simulink model "Shaddad_Perception"  (R2026b)
undefined symbols (not defined in the file): P, sens_per_prior_map, sens_per_prm, Ts
libraries: simulink x7, ros2lib x3, dspstat3 x1
settings Model: Creator=aomar  LastModifiedBy=aomar

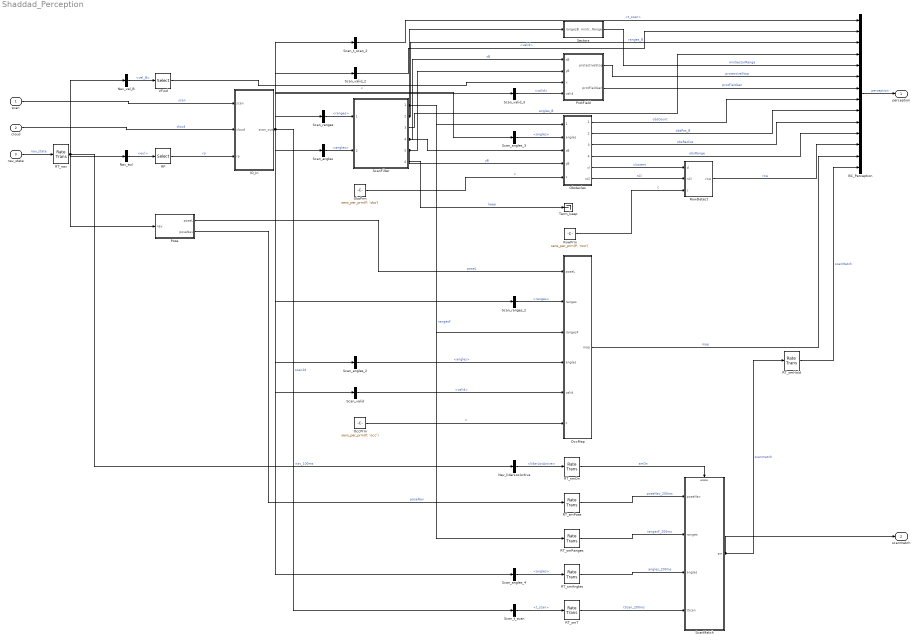
== system Shaddad_Perception ==
  scan : Inport  OutDataTypeStr=Bus: Bus_LidarScanRaw  SampleTime=Ts.lidar  BusOutputAsStruct=on
  cloud : Inport  Port=2  OutDataTypeStr=Bus: Bus_LidarCloudRaw  SampleTime=Ts.lidar  BusOutputAsStruct=on
  nav_state : Inport  Port=3  OutDataTypeStr=Bus: Bus_NavState  SampleTime=Ts.nav  BusOutputAsStruct=on
  BC_Perception : BusCreator  Inputs=14  OutDataTypeStr=Bus: Bus_Perception  NonVirtualBus=on
      settings: InheritFromInputs=off
  IO_In : Subsystem  Variant=on
  Nav_eul : BusSelector  OutputSignals=eul
  Nav_lidarLocActive : BusSelector  OutputSignals=lidarLocActive
  Nav_vel_B : BusSelector  OutputSignals=vel_B
  ObsPrm : Constant  Value=sens_per_prm(P, 'obs')
  Obstacles : MATLAB Function  TreatAsAtomicUnit=on
  OccMap : MATLAB Function  TreatAsAtomicUnit=on
  OccPrm : Constant  Value=sens_per_prm(P, 'occ')
  Pose : Subsystem  Description=poseL = [x + rLx cos psi - rLy sin psi, y + rLx sin psi + rLy cos psi, psi + psiL]; poseNav = [x y psi].
  ProtField : Subsystem  Description=Protective field (sensors spec 3.7): length protL0 + protKv |v|, width protW; the front field ahead of x = protXF (front of the body or of the fitted implement) when v > -protVBoth, the rear field behind x = protXR (rear of the body or implement) when v < protVBoth (both at standstill); a field stops when any kept point lies inside. Scan lost or stale (critfix R-02): on an invalid scan the last valid field result is held for up to protNStale scans, then protectiveStop is true until a valid scan arrives; true from the start until the first valid scan.
  RP : Selector  InputPortWidth=3  IndexOptions=Index vector (dialog)  Indices=[3 2]  OutputSizes=1
  RT_nav : RateTransition  OutPortSampleTime=Ts.perception
  RT_smAngles : RateTransition  OutPortSampleTime=Ts.scanmatch
  RT_smHold : RateTransition  InitialCondition=P.ic.Bus_ScanMatchMeas  OutPortSampleTime=Ts.perception
  RT_smOn : RateTransition  OutPortSampleTime=Ts.scanmatch
  RT_smPose : RateTransition  OutPortSampleTime=Ts.scanmatch
  RT_smRanges : RateTransition  OutPortSampleTime=Ts.scanmatch
  RT_smT : RateTransition  OutPortSampleTime=Ts.scanmatch
  RowDetect : MATLAB Function  TreatAsAtomicUnit=on
  RowPrm : Constant  Value=sens_per_prm(P, 'row')
  ScanFilter : Subsystem  ReferencedSubsystem=sens_scan_filter
  ScanMatch : Subsystem  Description=Enabled at 0.2 s while nav_state.lidarLocActive (D55); output reset to P.ic.Bus_ScanMatchMeas (valid false) while disabled.  TreatAsAtomicUnit=on
  Scan_angles : BusSelector  OutputSignals=angles
  Scan_angles_2 : BusSelector  OutputSignals=angles
  Scan_angles_3 : BusSelector  OutputSignals=angles
  Scan_angles_4 : BusSelector  OutputSignals=angles
  Scan_ranges : BusSelector  OutputSignals=ranges
  Scan_ranges_2 : BusSelector  OutputSignals=ranges
  Scan_t_scan : BusSelector  OutputSignals=t_scan
  Scan_t_scan_2 : BusSelector  OutputSignals=t_scan
  Scan_valid : BusSelector  OutputSignals=valid
  Scan_valid_2 : BusSelector  OutputSignals=valid
  Scan_valid_3 : BusSelector  OutputSignals=valid
  Sectors : Subsystem  Description=8 x 45 deg sector minima of ranges_B (sector j covers sensor beams -22 + 45 (j-1) ... +22 + 45 (j-1) deg, CCW): NaN -> Inf, Selector P.sensors.per.secIdx, Reshape [45 8], dspstat3/Minimum per column, empty sector -> NaN.
  Term_keep : Terminator
  VFwd : Selector  InputPortWidth=3  IndexOptions=Index vector (dialog)  Indices=1  OutputSizes=1
  perception : Outport  OutDataTypeStr=Bus: Bus_Perception  SampleTime=Ts.perception  BusOutputAsStruct=on
  scanmatch : Outport  Port=2  OutDataTypeStr=Bus: Bus_ScanMatchMeas  SampleTime=Ts.scanmatch  BusOutputAsStruct=on
  wires:
  scan/1 -> IO_In/1(scan)  "scan"
  cloud/1 -> IO_In/2(cloud)  "cloud"
  nav_state/1 -> RT_nav/1  "nav_state"
  RT_nav/1 -> Nav_lidarLocActive/1, Nav_vel_B/1, Pose/1(nav), Nav_eul/1  "nav_100ms"
  Nav_vel_B/1 -> VFwd/1  "<vel_B>"
  Nav_eul/1 -> RP/1  "<eul>"
  VFwd/1 -> ProtField/3(v)  "v"
  RP/1 -> IO_In/3(rp)  "rp"
  Pose/1(poseL) -> OccMap/1(poseL)  "poseL"
  Pose/2(poseNav) -> RT_smPose/1  "poseNav"
  IO_In/1(scan_out) -> Scan_t_scan/1, Scan_angles_4/1, Scan_valid/1, Scan_angles_2/1, Scan_ranges_2/1, Scan_t_scan_2/1, Scan_valid_2/1, Scan_valid_3/1, Scan_angles/1, Scan_ranges/1, Scan_angles_3/1  "scan2d"
  Scan_ranges/1 -> ScanFilter/1  "<ranges>"
  Scan_angles/1 -> ScanFilter/2  "<angles>"
  Scan_t_scan_2/1 -> BC_Perception/1  "<t_scan>"
  Scan_valid_2/1 -> BC_Perception/2  "<valid>"
  Scan_angles_2/1 -> OccMap/4(angles)  "<angles>"
  Scan_valid/1 -> OccMap/5(valid)  "<valid>"
  ObsPrm/1 -> Obstacles/5(c)  "c"
  OccPrm/1 -> OccMap/6(c)  "c"
  ScanFilter/3 -> BC_Perception/4  "angles_B"
  ScanFilter/6 -> Term_keep/1  "keep"
  Scan_valid_3/1 -> ProtField/4(valid)  "<valid>"
  Scan_angles_3/1 -> Obstacles/2(angles)  "<angles>"
  Scan_ranges_2/1 -> OccMap/2(ranges)  "<ranges>"
  Nav_lidarLocActive/1 -> RT_smOn/1  "<lidarLocActive>"
  Scan_angles_4/1 -> RT_smAngles/1  "<angles>"
  Scan_t_scan/1 -> RT_smT/1  "<t_scan>"
  RowPrm/1 -> RowDetect/3(c)  "c"
  RT_smOn/1 -> ScanMatch/Enable  "smOn"
  RT_smPose/1 -> ScanMatch/1(poseNav)  "poseNav_200ms"
  RT_smRanges/1 -> ScanMatch/2(ranges)  "rangesF_200ms"
  RT_smAngles/1 -> ScanMatch/3(angles)  "angles_200ms"
  RT_smT/1 -> ScanMatch/4(tScan)  "tScan_200ms"
  Obstacles/1(obsCount) -> BC_Perception/8  "obsCount"
  Obstacles/2(obsPos) -> BC_Perception/9  "obsPos_B"
  Obstacles/3(obsRadius) -> BC_Perception/10  "obsRadius"
  Obstacles/4(obsRange) -> BC_Perception/11  "obsRange"
  Obstacles/5(cl) -> RowDetect/1(cl)  "clusters"
  Obstacles/6(nCl) -> RowDetect/2(nCl)  "nCl"
  OccMap/1(map) -> BC_Perception/13  "map"
  Sectors/1(minSectorRange) -> BC_Perception/5  "minSectorRange"
  ProtField/1(protectiveStop) -> BC_Perception/6  "protectiveStop"
  ProtField/2(protFieldLen) -> BC_Perception/7  "protFieldLen"
  RowDetect/1(row) -> BC_Perception/12  "row"
  ScanMatch/1(sm) -> RT_smHold/1, scanmatch/1  "scanmatch"
  RT_smHold/1 -> BC_Perception/14  "scanMatch"
  BC_Perception/1 -> perception/1  "perception"
  ScanFilter/1 -> RT_smRanges/1, OccMap/3(rangesF), Obstacles/1(rangesF)  "rangesF"
  ScanFilter/5 -> ProtField/2(yB), Obstacles/4(yB)  "yB"
  ScanFilter/4 -> ProtField/1(xB), Obstacles/3(xB)  "xB"
  ScanFilter/2 -> Sectors/1(rangesB), BC_Perception/3  "ranges_B"

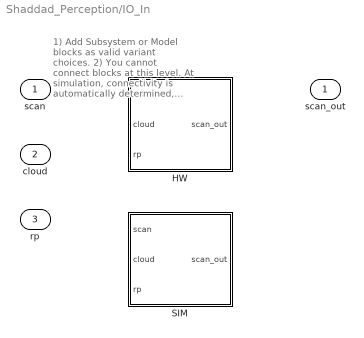
== system Shaddad_Perception/IO_In ==
  note: 1) Add Subsystem or Model blocks as valid variant choices.
      | 2) You cannot connect blocks at this level. At simulation, connectivity is automatically
      | determined, based on the active variant and port name matching.
  scan : Inport
  cloud : Inport  Port=2
  rp : Inport  Port=3
  HW : Subsystem  Description=HW (VC_TARGET == 1): ros2lib/Subscribe /ouster/points (sensor_msgs/PointCloud2, 0.1 s) -> ros2lib/Read Point Cloud [32 1024] organised -> MATLAB Function sens_lidar_cloud2scan -> Bus_LidarScanRaw (t_scan = ROS time at reception, ros2lib/Current Time).  VariantControl=VC_TARGET == 1
  SIM : Subsystem  Description=SIM (VC_TARGET == 0): Subsystem Reference sens_acq_lidar (scan source Variant VC_LIDAR).  VariantControl=VC_TARGET == 0
  scan_out : Outport

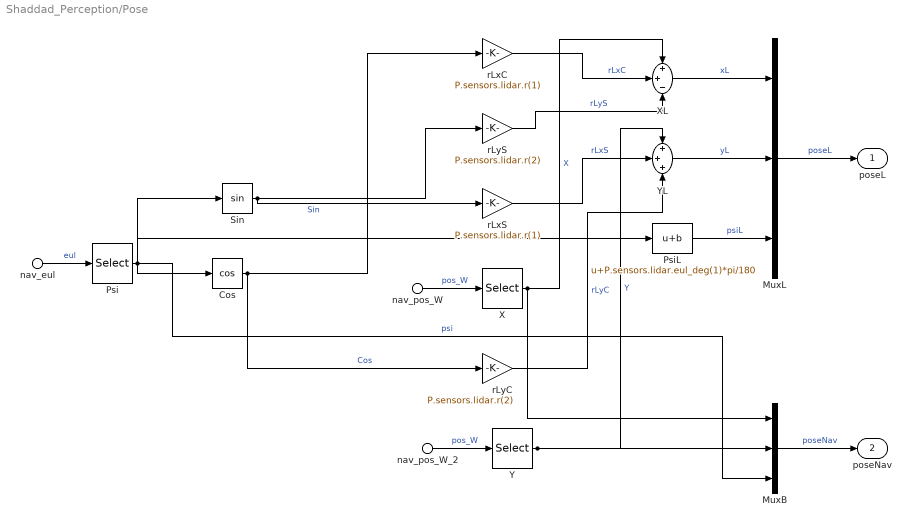
== system Shaddad_Perception/Pose ==
  nav_pos_W : Inport  PortName=nav  Element=pos_W
  nav_pos_W_2 : Inport  PortName=nav  Element=pos_W
  nav_eul : Inport  PortName=nav  Element=eul
  Cos : Trigonometry  Operator=cos
  MuxB : Mux  Inputs=3
  MuxL : Mux  Inputs=3
  Psi : Selector  InputPortWidth=3  IndexOptions=Index vector (dialog)  Indices=1  OutputSizes=1
  PsiL : Bias  Bias=P.sensors.lidar.eul_deg(1)*pi/180  SaturateOnIntegerOverflow=off
  Sin : Trigonometry
  X : Selector  InputPortWidth=3  IndexOptions=Index vector (dialog)  Indices=1  OutputSizes=1
  XL : Sum  Inputs=++-
  Y : Selector  InputPortWidth=3  IndexOptions=Index vector (dialog)  Indices=2  OutputSizes=1
  YL : Sum  Inputs=+++
  rLxC : Gain  Gain=P.sensors.lidar.r(1)
  rLxS : Gain  Gain=P.sensors.lidar.r(1)
  rLyC : Gain  Gain=P.sensors.lidar.r(2)
  rLyS : Gain  Gain=P.sensors.lidar.r(2)
  poseL : Outport
  poseNav : Outport  Port=2
  wires:
  nav_eul/1 -> Psi/1  "eul"
  Psi/1 -> MuxB/3, Sin/1, PsiL/1, Cos/1  "psi"
  Cos/1 -> rLxC/1, rLyC/1  "Cos"
  Sin/1 -> rLyS/1, rLxS/1  "Sin"
  nav_pos_W/1 -> X/1  "pos_W"
  nav_pos_W_2/1 -> Y/1  "pos_W"
  rLxC/1 -> XL/2  "rLxC"
  rLxS/1 -> YL/2  "rLxS"
  rLyC/1 -> YL/3  "rLyC"
  X/1 -> XL/1, MuxB/1  "X"
  XL/1 -> MuxL/1  "xL"
  YL/1 -> MuxL/2  "yL"
  PsiL/1 -> MuxL/3  "psiL"
  MuxL/1 -> poseL/1  "poseL"
  MuxB/1 -> poseNav/1  "poseNav"
  rLyS/1 -> XL/3  "rLyS"
  Y/1 -> YL/1, MuxB/2  "Y"

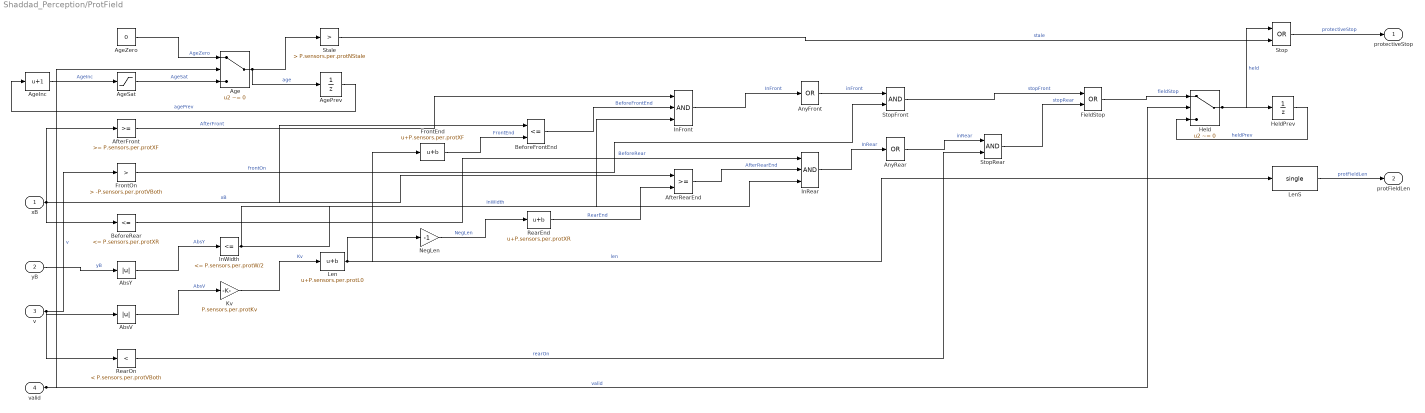
== system Shaddad_Perception/ProtField ==
  xB : Inport
  yB : Inport  Port=2
  v : Inport  Port=3
  valid : Inport  Port=4
  AbsV : Abs  SaturateOnIntegerOverflow=off
  AbsY : Abs  SaturateOnIntegerOverflow=off
  AfterFront : simulink/Logic and Bit Operations/Compare To Constant  relop=>=  const=P.sensors.per.protXF  OutDataTypeStr=boolean
  AfterRearEnd : RelationalOperator  OutDataTypeStr=boolean  RndMeth=Simplest  InputSameDT=off
  Age : Switch  Criteria=u2 ~= 0  OutDataTypeStr=double  SaturateOnIntegerOverflow=off  InputSameDT=off
  AgeInc : Bias  Bias=1  SaturateOnIntegerOverflow=off
  AgePrev : UnitDelay  InitialCondition=P.sensors.per.protNStale + 1  SampleTime=Ts.perception
  AgeSat : Saturate  UpperLimit=P.sensors.per.protNStale + 1  LowerLimit=0
  AgeZero : Constant  Value=0
  AnyFront : Logic  Operator=OR  Inputs=1  AllPortsSameDT=off  OutDataTypeStr=boolean
  AnyRear : Logic  Operator=OR  Inputs=1  AllPortsSameDT=off  OutDataTypeStr=boolean
  BeforeFrontEnd : RelationalOperator  Operator=<=  OutDataTypeStr=boolean  RndMeth=Simplest  InputSameDT=off
  BeforeRear : simulink/Logic and Bit Operations/Compare To Constant  relop=<=  const=P.sensors.per.protXR  OutDataTypeStr=boolean
  FieldStop : Logic  Operator=OR  AllPortsSameDT=off  OutDataTypeStr=boolean
  FrontEnd : Bias  Bias=P.sensors.per.protXF  SaturateOnIntegerOverflow=off
  FrontOn : simulink/Logic and Bit Operations/Compare To Constant  relop=>  const=-P.sensors.per.protVBoth  OutDataTypeStr=boolean
  Held : Switch  Criteria=u2 ~= 0  OutDataTypeStr=boolean  SaturateOnIntegerOverflow=off  InputSameDT=off
  HeldPrev : UnitDelay  InitialCondition=true  SampleTime=Ts.perception
  InFront : Logic  Inputs=3  AllPortsSameDT=off  OutDataTypeStr=boolean
  InRear : Logic  Inputs=3  AllPortsSameDT=off  OutDataTypeStr=boolean
  InWidth : simulink/Logic and Bit Operations/Compare To Constant  relop=<=  const=P.sensors.per.protW/2  OutDataTypeStr=boolean
  Kv : Gain  Gain=P.sensors.per.protKv
  Len : Bias  Bias=P.sensors.per.protL0  SaturateOnIntegerOverflow=off
  LenS : DataTypeConversion  OutDataTypeStr=single  RndMeth=Nearest  SaturateOnIntegerOverflow=off
  NegLen : Gain  Gain=-1
  RearEnd : Bias  Bias=P.sensors.per.protXR  SaturateOnIntegerOverflow=off
  RearOn : simulink/Logic and Bit Operations/Compare To Constant  relop=<  const=P.sensors.per.protVBoth  OutDataTypeStr=boolean
  Stale : simulink/Logic and Bit Operations/Compare To Constant  relop=>  const=P.sensors.per.protNStale  OutDataTypeStr=boolean
  Stop : Logic  Operator=OR  AllPortsSameDT=off  OutDataTypeStr=boolean
  StopFront : Logic  AllPortsSameDT=off  OutDataTypeStr=boolean
  StopRear : Logic  AllPortsSameDT=off  OutDataTypeStr=boolean
  protectiveStop : Outport
  protFieldLen : Outport  Port=2
  wires:
  xB/1 -> BeforeFrontEnd/1, AfterFront/1, AfterRearEnd/1, BeforeRear/1  "xB"
  yB/1 -> AbsY/1  "yB"
  v/1 -> FrontOn/1, RearOn/1, AbsV/1  "v"
  valid/1 -> Age/2, Held/2  "valid"
  AgeInc/1 -> AgeSat/1  "AgeInc"
  AgeZero/1 -> Age/1  "AgeZero"
  AgeSat/1 -> Age/3  "AgeSat"
  AfterFront/1 -> InFront/1  "AfterFront"
  FrontOn/1 -> StopFront/2  "frontOn"
  BeforeRear/1 -> InRear/1  "BeforeRear"
  AbsY/1 -> InWidth/1  "AbsY"
  AbsV/1 -> Kv/1  "AbsV"
  RearOn/1 -> StopRear/2  "rearOn"
  InWidth/1 -> InFront/3, InRear/3  "InWidth"
  Kv/1 -> Len/1  "Kv"
  Age/1 -> Stale/1, AgePrev/1  "age"
  Stale/1 -> Stop/2  "stale"
  AgePrev/1 -> AgeInc/1  "agePrev"
  Len/1 -> FrontEnd/1, LenS/1, NegLen/1  "len"
  NegLen/1 -> RearEnd/1  "NegLen"
  FrontEnd/1 -> BeforeFrontEnd/2  "FrontEnd"
  BeforeFrontEnd/1 -> InFront/2  "BeforeFrontEnd"
  RearEnd/1 -> AfterRearEnd/2  "RearEnd"
  InFront/1 -> AnyFront/1  "InFront"
  AfterRearEnd/1 -> InRear/2  "AfterRearEnd"
  AnyFront/1 -> StopFront/1  "inFront"
  InRear/1 -> AnyRear/1  "InRear"
  StopFront/1 -> FieldStop/1  "stopFront"
  AnyRear/1 -> StopRear/1  "inRear"
  StopRear/1 -> FieldStop/2  "stopRear"
  FieldStop/1 -> Held/1  "fieldStop"
  Held/1 -> Stop/1, HeldPrev/1  "held"
  Stop/1 -> protectiveStop/1  "protectiveStop"
  HeldPrev/1 -> Held/3  "heldPrev"
  LenS/1 -> protFieldLen/1  "protFieldLen"

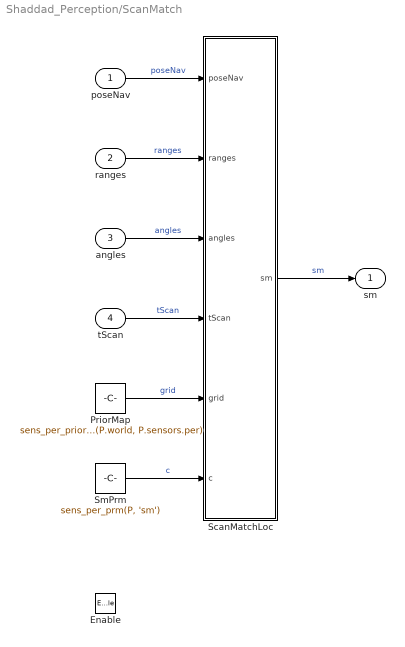
== system Shaddad_Perception/ScanMatch ==
  poseNav : Inport
  ranges : Inport  Port=2
  angles : Inport  Port=3
  tScan : Inport  Port=4
  Enable : EnablePort
  PriorMap : Constant  Value=sens_per_prior_map(P.world, P.sensors.per)  VectorParams1D=off  OutDataTypeStr=boolean
  ScanMatchLoc : MATLAB Function  TreatAsAtomicUnit=on
  SmPrm : Constant  Value=sens_per_prm(P, 'sm')
  sm : Outport  OutDataTypeStr=Bus: Bus_ScanMatchMeas  OutputWhenDisabled=reset  InitialOutput=P.ic.Bus_ScanMatchMeas
  wires:
  poseNav/1 -> ScanMatchLoc/1(poseNav)  "poseNav"
  ranges/1 -> ScanMatchLoc/2(ranges)  "ranges"
  angles/1 -> ScanMatchLoc/3(angles)  "angles"
  tScan/1 -> ScanMatchLoc/4(tScan)  "tScan"
  PriorMap/1 -> ScanMatchLoc/5(grid)  "grid"
  SmPrm/1 -> ScanMatchLoc/6(c)  "c"
  ScanMatchLoc/1(sm) -> sm/1  "sm"

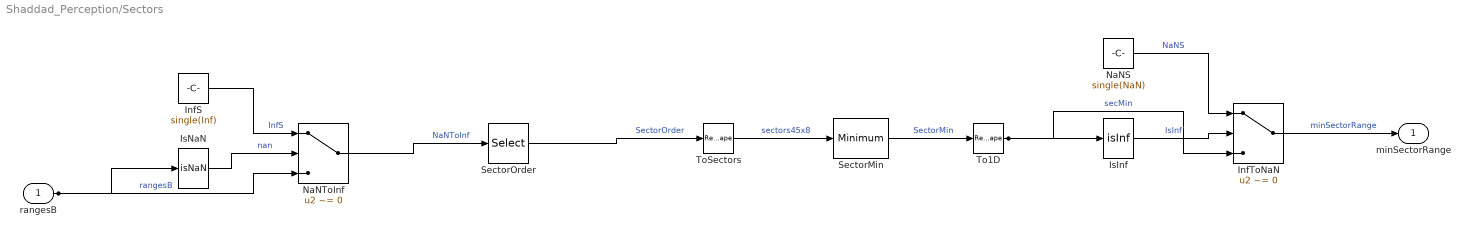
== system Shaddad_Perception/Sectors ==
  rangesB : Inport
  InfS : Constant  Value=single(Inf)  OutDataTypeStr=single
  InfToNaN : Switch  Criteria=u2 ~= 0  SaturateOnIntegerOverflow=off  InputSameDT=off
  IsInf : RelationalOperator  Operator=isInf  OutDataTypeStr=boolean  RndMeth=Simplest  InputSameDT=off
  IsNaN : RelationalOperator  Operator=isNaN  OutDataTypeStr=boolean  RndMeth=Simplest  InputSameDT=off
  NaNS : Constant  Value=single(NaN)  OutDataTypeStr=single
  NaNToInf : Switch  Criteria=u2 ~= 0  SaturateOnIntegerOverflow=off  InputSameDT=off
  SectorMin : dspstat3/Minimum  operation=minimum  fcn=Value  indexBase=One  operateOver=Each column  Dimension=1  InputProcessing=Columns as channels (frame based)  reset=None  roiEnable=off  roiType=Rectangles  roiPortion=Entire ROI  roiOutput=Individual statistics for each ROI  roiFlag=off  roundingMode=Floor  overflowMode=off
  SectorOrder : Selector  InputPortWidth=P.sensors.lidar.nBeams  IndexOptions=Index vector (dialog)  Indices=P.sensors.per.secIdx  OutputSizes=1
  To1D : Reshape
  ToSectors : Reshape  OutputDimensionality=Customize  OutputDimensions=[P.sensors.per.secLen P.sensors.per.nSectors]
  minSectorRange : Outport
  wires:
  rangesB/1 -> IsNaN/1, NaNToInf/3  "rangesB"
  InfS/1 -> NaNToInf/1  "InfS"
  IsNaN/1 -> NaNToInf/2  "nan"
  NaNToInf/1 -> SectorOrder/1  "NaNToInf"
  SectorOrder/1 -> ToSectors/1  "SectorOrder"
  ToSectors/1 -> SectorMin/1  "sectors45x8"
  SectorMin/1 -> To1D/1  "SectorMin"
  To1D/1 -> InfToNaN/3, IsInf/1  "secMin"
  NaNS/1 -> InfToNaN/1  "NaNS"
  IsInf/1 -> InfToNaN/2  "IsInf"
  InfToNaN/1 -> minSectorRange/1  "minSectorRange"

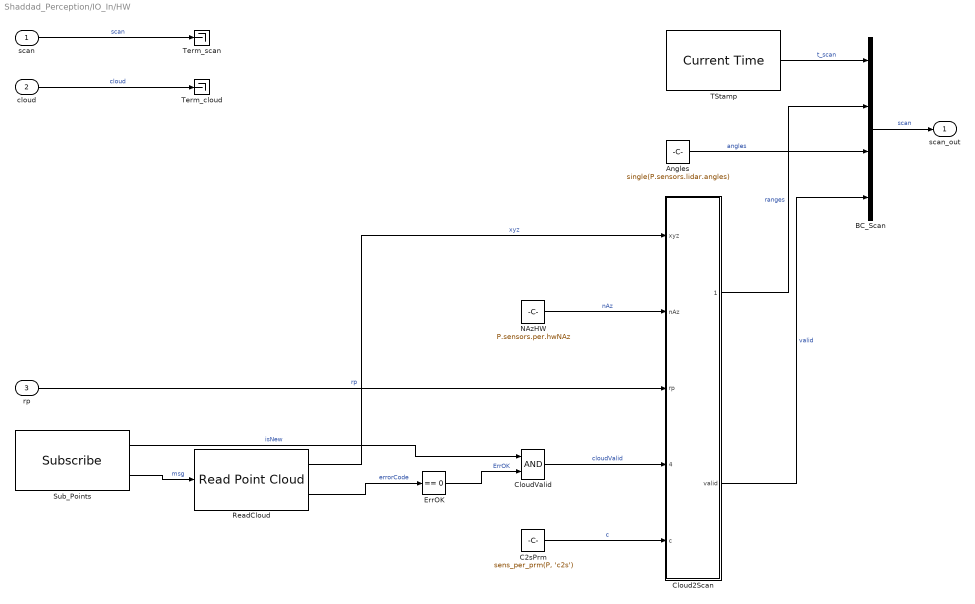
== system Shaddad_Perception/IO_In/HW ==
  scan : Inport
  cloud : Inport  Port=2
  rp : Inport  Port=3
  Angles : Constant  Value=single(P.sensors.lidar.angles)  OutDataTypeStr=single  SampleTime=Ts.lidar
  BC_Scan : BusCreator  Inputs=4  OutDataTypeStr=Bus: Bus_LidarScanRaw  NonVirtualBus=on
      settings: InheritFromInputs=off
  C2sPrm : Constant  Value=sens_per_prm(P, 'c2s')
  Cloud2Scan : MATLAB Function  TreatAsAtomicUnit=on
  CloudValid : Logic  AllPortsSameDT=off  OutDataTypeStr=boolean
  ErrOK : simulink/Logic and Bit Operations/Compare To Constant  relop===  const=0  OutDataTypeStr=boolean
  NAzHW : Constant  Value=P.sensors.per.hwNAz
  ReadCloud : ros2lib/Read Point Cloud  MaximumPointCloudSize=P.sensors.lidar.cloudSize  PreserveStructure=on  ShowRGBOutput=off  ShowIntensityOutput=off  ShowErrorCodeOutput=on  VariableSizeOutputs=off
  Sub_Points : ros2lib/Subscribe  topicSource=Specify your own  topic=/ouster/points  messageType=sensor_msgs/PointCloud2  SubscriberMode=At sample time  sampleTime=Ts.lidar  CallbackGroupType=Default  CallbackGroupName=callback_group_1  QOSHistory=Keep last  QOSDepth=10  QOSReliability=Reliable  QOSDurability=Volatile  QOSDeadline=Inf  QOSLifespan=Inf  QOSLiveliness=Automatic  QOSLeaseDuration=Inf  QOSAvoidROSNamespaceConventions=off
  TStamp : ros2lib/Current Time  OutputFormat=double  SampleTime=Ts.lidar  ModelName=untitled
  Term_cloud : Terminator
  Term_scan : Terminator
  scan_out : Outport
  wires:
  scan/1 -> Term_scan/1  "scan"
  cloud/1 -> Term_cloud/1  "cloud"
  rp/1 -> Cloud2Scan/3(rp)  "rp"
  Sub_Points/1 -> CloudValid/1  "isNew"
  Sub_Points/2 -> ReadCloud/1  "msg"
  ReadCloud/1 -> Cloud2Scan/1(xyz)  "xyz"
  ReadCloud/2 -> ErrOK/1  "errorCode"
  ErrOK/1 -> CloudValid/2  "ErrOK"
  NAzHW/1 -> Cloud2Scan/2(nAz)  "nAz"
  CloudValid/1 -> Cloud2Scan/4(cloudValid)  "cloudValid"
  C2sPrm/1 -> Cloud2Scan/5(c)  "c"
  Angles/1 -> BC_Scan/3  "angles"
  Cloud2Scan/1(ranges) -> BC_Scan/2  "ranges"
  Cloud2Scan/2(valid) -> BC_Scan/4  "valid"
  TStamp/1 -> BC_Scan/1  "t_scan"
  BC_Scan/1 -> scan_out/1  "scan"

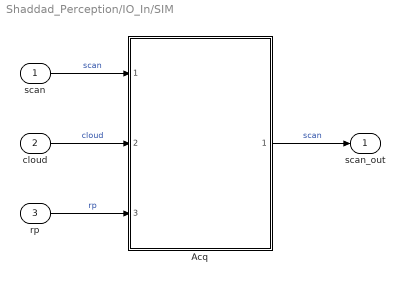
== system Shaddad_Perception/IO_In/SIM ==
  scan : Inport
  cloud : Inport  Port=2
  rp : Inport  Port=3
  Acq : Subsystem  ReferencedSubsystem=sens_acq_lidar
  scan_out : Outport
  wires:
  scan/1 -> Acq/1  "scan"
  cloud/1 -> Acq/2  "cloud"
  rp/1 -> Acq/3  "rp"
  Acq/1 -> scan_out/1  "scan"

== matlab function Shaddad_Perception/IO_In/HW/Cloud2Scan ==
  settings: description=Cloud -> 360-beam height-band scan (sensors spec 3.4 / F4): subsystems/sensors/sens_lidar_cloud2scan.m; constants on input 5 (sens_per_prm(P, 'c2s'))
  data: xyz input; ranges output; nAz input; rp input; cloudValid input; c input; valid output
function [ranges, valid] = fcn(xyz, nAz, rp, cloudValid, c)
%#codegen
[ranges, valid] = sens_lidar_cloud2scan(xyz, nAz, rp, cloudValid, c);

== matlab function Shaddad_Perception/OccMap ==
  settings: description=Rolling 30 x 30 m occupancy grid in the TEB MapInfo format (sensors spec 3.7 / F8): subsystems/sensors/sens_occmap_update.m; constants on input 6 (sens_per_prm(P, 'occ'))
  data: poseL input; map output Bus: Bus_TebMapInfo; ranges input; rangesF input; angles input; valid input; c input
function map = fcn(poseL, ranges, rangesF, angles, valid, c)
%#codegen
map = sens_occmap_update(poseL, ranges, rangesF, angles, valid, c);

== matlab function Shaddad_Perception/Obstacles ==
  settings: description=Obstacle segmentation loop (sensors spec 3.7 / F9, D59): subsystems/sensors/sens_obstacle_extract.m; constants on input 5 (sens_per_prm(P, 'obs'))
  data: rangesF input; obsCount output; angles input; xB input; yB input; c input; obsPos output; obsRadius output; obsRange output; cl output; nCl output
function [obsCount, obsPos, obsRadius, obsRange, cl, nCl] = fcn(rangesF, angles, xB, yB, c)
%#codegen
[obsCount, obsPos, obsRadius, obsRange, cl, nCl] = sens_obstacle_extract(rangesF, angles, xB, yB, c);

== matlab function Shaddad_Perception/RowDetect ==
  settings: description=Row detection, RANSAC line per side (sensors spec 3.7 / F10): subsystems/sensors/sens_row_detect.m; constants on input 3 (sens_per_prm(P, 'row'))
  data: cl input; row output Bus: Bus_RowFeature; nCl input; c input
function row = fcn(cl, nCl, c)
%#codegen
row = sens_row_detect(cl, nCl, c);

== matlab function Shaddad_Perception/ScanMatch/ScanMatchLoc ==
  settings: description=Scan-to-prior-map localisation with matchScansGrid (sensors spec 3.7 / F11, D55): subsystems/sensors/sens_scanmatch_loc.m; prior map on input 5 (sens_per_prior_map(P.world, P.sensors.per)), constants on input 6 (sens_per_prm(P, 'sm'))
  data: poseNav input; sm output Bus: Bus_ScanMatchMeas; ranges input; angles input; tScan input; grid input; c input
function sm = fcn(poseNav, ranges, angles, tScan, grid, c)
%#codegen
sm = sens_scanmatch_loc(poseNav, ranges, angles, tScan, grid, c);
